simulink model "Stateflow_Transmission_Logic"  (R2026b)
settings: Solver=VariableStepAuto
libraries: simulink x1
settings Model: Creator=maryliya  LastModifiedBy=maryliya

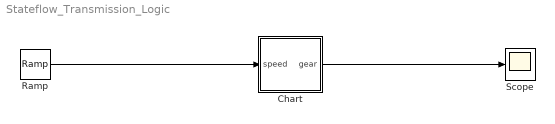
== system Stateflow_Transmission_Logic ==
  Chart : Stateflow chart  TreatAsAtomicUnit=on
  Ramp : simulink/Sources/Ramp  slope=10  start=0  InitialOutput=0
  Scope : Scope
      settings: ActiveDisplayYMinimum=0.875  ActiveDisplayYMaximum=2.125
  wires:
  Ramp/1 -> Chart/1(speed)
  Chart/1(gear) -> Scope/1

== stateflow chart Stateflow_Transmission_Logic/Chart ==
  state Gear1
    gear=1
  state Gear2
    gear=2
  Gear1 -> Gear2 : [speed>40]
  Gear2 -> Gear1 : [speed<=35]
  (default) -> Gear1
  data: speed input; gear output
